simulink model "BallRegulator"  (R2026a)
settings: Solver=VariableStepAuto
libraries: fl_lib x6, nesl_utility x4, SimscapeFluids_lib x1, slpidlib x1
settings Model: Creator=lucas  LastModifiedBy=lucas

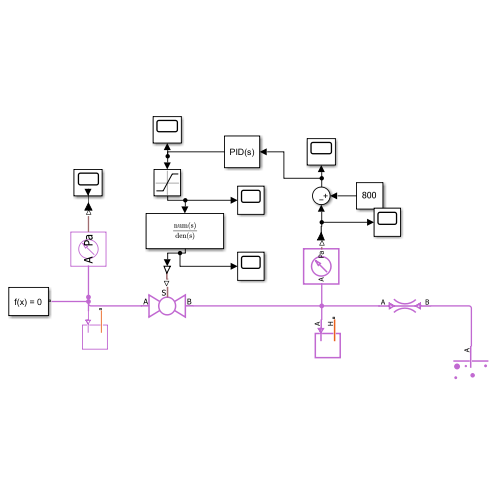
[thumbnail: Simulink's stored preview of the top-level diagram]
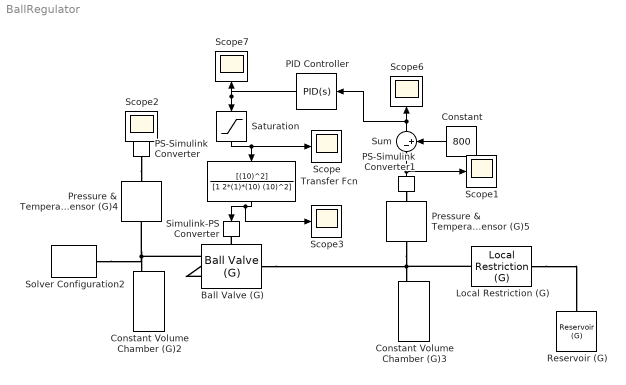
== system BallRegulator ==
  Ball Valve (G) : SimscapeFluids_lib/Gas/Valves & Orifices/Flow Control Valves/Ball Valve (G)  valve_parameterization=fluids.gas.valves_orifices.flow_control_valves.enum.OrificeParameterization.Geometry  opening_characteristic=fluids.gas.valves_orifices.flow_control_valves.enum.BallValveSpec.OverlappingCircles  Cv_max=4  rotation_Cv_TLU=pi / 2 * (0 : 0.1 : 1) rad  Cv_TLU=[1e-06, .0725, .1437, .2375, .35, .5375, .875, 1.3125, 2.125, 3.25, 4]  xT_Cv=0.7  Kv_max=3.6  rotation_Kv_TLU=pi / 2 * (0 : 0.1 : 1) rad  Kv_TLU=[1e-06, .0653, .1293, .2137, .315, .4838, .7875, 1.1813, 1.8381, 2.8112, 3.6]  xT_Kv=0.7  C_max=12 l/(bar*s)  B_crit_C=0.3  rotation_C_TLU=pi / 2 * (0 : 0.1 : 1) rad  C_TLU=[1e-05, .2175, .4312, .7125, 1.05, 1.6125, 2.625, 3.9375, 6.375, 9.75, 12] l/(bar*s)  B_crit_TLU=0.3 * ones(1, 11)  m=0.5  T_ref_C=293.15 K  rho_ref_C=1.185 kg/m^3  rotation_area_TLU=pi / 2 * (0 : 0.1 : 1) rad  area_TLU=[1e-10, 45, 90, 135, 180, 225, 270, 315, 360, 405, 450] mm^2  area_ball=pi * ((1/3) ^ 2) in^2  area=pi * ((1/2) ^ 2) in^2  Cd=0.64  leakage_fraction=1e-6  B_lam=0.999
  Constant : Constant  Value=800
  Constant Volume Chamber (G)2 : fl_lib/Gas/Elements/Constant Volume Chamber (G)  volume=0.01 m^3  num_ports=foundation.enum.num_ports.one  area_A=0.01 m^2  area_B=0.01 m^2  area_C=0.01 m^2  area_D=0.01 m^2  p_I_specify=on  p_I_priority=High  p_I=4500 psi  p_I_nominal_specify=off  p_I_nominal_value=1  p_I_nominal_unit=MPa  T_I_specify=off  T_I_priority=High  T_I=293.15 K  T_I_nominal_specify=off  T_I_nominal_value=1  T_I_nominal_unit=K  rho_I_specify=off  rho_I_priority=None  rho_I=1.2 kg/m^3  rho_I_nominal_specify=off  rho_I_nominal_value=1  rho_I_nominal_unit=kg/m^3
  Constant Volume Chamber (G)3 : fl_lib/Gas/Elements/Constant Volume Chamber (G)  volume=0.01 m^3  num_ports=foundation.enum.num_ports.one  area_A=0.01 m^2  area_B=0.01 m^2  area_C=0.01 m^2  area_D=0.01 m^2  p_I_specify=on  p_I_priority=Low  p_I=600 psi  p_I_nominal_specify=off  p_I_nominal_value=1  p_I_nominal_unit=MPa  T_I_specify=off  T_I_priority=High  T_I=293.15 K  T_I_nominal_specify=off  T_I_nominal_value=1  T_I_nominal_unit=K  rho_I_specify=off  rho_I_priority=None  rho_I=1.2 kg/m^3  rho_I_nominal_specify=off  rho_I_nominal_value=1  rho_I_nominal_unit=kg/m^3
  Local Restriction (G) : fl_lib/Gas/Elements/Local Restriction (G)  restriction_type=foundation.enum.restriction_type.fixed  restriction_area=pi * ((1/8)^2) in^2  min_area=1e-10 m^2  max_area=0.005 m^2  area=0.01 m^2  Cd=0.64  B_lam=0.999
  PID Controller : slpidlib/PID Controller  Controller=PID  Form=Parallel  TimeDomain=Continuous-time  UseExternalTs=off  SampleTime=-1  IntegratorMethod=Forward Euler  FilterMethod=Forward Euler  ControllerParametersSource=internal  P=0.005  I=0.01  UseKiTs=off  D=0.001  UseExternalDerivativeSource=off  N=100  UseFilter=on  TunerSelectOption=Transfer Function Based (PID Tuner App)  InitialConditionSource=internal  InitialConditionForIntegrator=0  InitialConditionForFilter=0  DifferentiatorICPrevScaledInput=0  ExternalReset=none  TrackingMode=off  Kt=1  LimitOutput=off  SatLimitsSource=internal  UpperSaturationLimit=inf  LowerSaturationLimit=-inf  LinearizeAsGain=on  AntiWindupMode=none  Kb=1  LimitIntegrator=off  UpperIntegratorSaturationLimit=inf  LowerIntegratorSaturationLimit=-inf  POutMin=[]  POutMax=[]  IOutMin=[]  IOutMax=[]  DOutMin=[]  DOutMax=[]  NOutMin=[]  NOutMax=[]  SumOutMin=[]  SumOutMax=[]  SaturationOutMin=[]  SaturationOutMax=[]  PParamMin=[]  PParamMax=[]  IParamMin=[]  IParamMax=[]  DParamMin=[]  DParamMax=[]  NParamMin=[]  NParamMax=[]  KbParamMin=[]  KbParamMax=[]  KtParamMin=[]  KtParamMax=[]  KbOutMin=[]  KbOutMax=[]  KtOutMin=[]  KtOutMax=[]  IntegratorOutMin=[]  IntegratorOutMax=[]  FilterOutMin=[]  FilterOutMax=[]  SumI1OutMin=[]  SumI1OutMax=[]  SumI2OutMin=[]  SumI2OutMax=[]  SumI3OutMin=[]  SumI3OutMax=[]  SumI4OutMin=[]  SumI4OutMax=[]  SumDOutMin=[]  SumDOutMax=[]  DifferentiatorOutMin=[]  DifferentiatorOutMax=[]  FilterDiffOutCoefMin=[]  FilterDiffOutCoefMax=[]  ReciprocalOutMin=[]  ReciprocalOutMax=[]  SumDenOutMin=[]  SumDenOutMax=[]  SumNumOutMin=[]  SumNumOutMax=[]  DivideOutMin=[]  DivideOutMax=[]  UdiffTsProdOutMin=[]  UdiffTsProdOutMax=[]  NTsProdOutMin=[]  NTsProdOutMax=[]  UintegralTsProdOutMin=[]  UintegralTsProdOutMax=[]  UngainTsProdOutMin=[]  UngainTsProdOutMax=[]  ClampingZeroOutDataTypeStr=Inherit: Inherit via back propagation  ClampingZeroOutMin=[]  ClampingZeroOutMax=[]  FilterDenConstantOutDataTypeStr=Inherit: Inherit via back propagation  FilterDenConstantOutMin=[]  FilterDenConstantOutMax=[]  PCopyOutDataTypeStr=Inherit: Inherit via back propagation  PCopyOutMin=[]  PCopyOutMax=[]  NCopyOutDataTypeStr=Inherit: Inherit via back propagation  NCopyOutMin=[]  NCopyOutMax=[]  IntegratorContinuousStateAttributes=''  IntegratorStateMustResolveToSignalObject=off  IntegratorRTWStateStorageClass=Auto  FilterContinuousStateAttributes=''  FilterStateMustResolveToSignalObject=off  FilterRTWStateStorageClass=Auto  ParallelPVariant=InternalParameters  IdealPVariant=Disabled  IVariant=InternalParameters  DVariant=InternalParameters  IntegratorVariant=Continuous  SatVariant=Disabled  AWVariant=Passthrough  PCopyVariant=Disabled  TRVariant=Disabled  FdbkBlocksVariant=Forward  IdealPFdbkVariant=Disabled  SatFdbkVariant=Disabled  DerivativeFilterVariant=ContFilter  NVariant=InternalParameters  NCopyVariant=Disabled  FilterICVariant=InternalICsFilter  IntegratorICVariant=InternalICs  ExternalResetVariant=Disabled  TRSumVariant=Passthrough  SumFdbkVariant=Disabled  SumVariant=Sum_PID  TsampFilterVariant=InternalTs  TsampNgainVariant=Passthrough  TsampIntegralVariant=Disabled_SignalSpec  ExternalSaturationOutDataTypeStr=Inherit: Same as second input  DerivativeSourceVariant=ErrorSignal  PreIntVariant=InternalPreInt
  PS-Simulink Converter : nesl_utility/PS-Simulink Converter  PhysicalDomain=network_engine_domain  SubClassName=ps_output  LeftPortType=input  RightPortType=output  PseudoPeriodic=off  Frequencies=[]  VectorFormat=inherit  Unit=psi  AffineConversion=off
  PS-Simulink Converter1 : nesl_utility/PS-Simulink Converter  PhysicalDomain=network_engine_domain  SubClassName=ps_output  LeftPortType=input  RightPortType=output  PseudoPeriodic=off  Frequencies=[]  VectorFormat=inherit  Unit=psi  AffineConversion=off
  Pressure & Temperature Sensor (G)4 : fl_lib/Gas/Sensors/Pressure & Temperature Sensor (G)  reference=foundation.enum.MeasurementReference.absolute  pressure=true  pressure_spec=foundation.enum.PressureMeasementSpec.Absolute  temperature=false
  Pressure & Temperature Sensor (G)5 : fl_lib/Gas/Sensors/Pressure & Temperature Sensor (G)  reference=foundation.enum.MeasurementReference.absolute  pressure=true  pressure_spec=foundation.enum.PressureMeasementSpec.Absolute  temperature=false
  Reservoir (G) : fl_lib/Gas/Elements/Reservoir (G)  pressure_input=false  pressure_spec=foundation.enum.pressure_spec.atmospheric  reservoir_pressure=0.101325 MPa  temperature_input=false  reservoir_temperature=293.15 K  area_A=0.01 m^2  input_error_spec=foundation.enum.input_range_error.warn
  Saturation : Saturate  UpperLimit=pi/2  LowerLimit=0
  Scope{,1..3,6..7} (6 alike) : Scope
      Scope settings: ActiveDisplayYMinimum=-0.73133757213653627  ActiveDisplayYMaximum=2.7321181317120371
      Scope1 settings: ActiveDisplayYMinimum=309.130990645238  ActiveDisplayYMaximum=966.57527246233519  DataLoggingVariableName=ScopeData2
      Scope2 settings: ActiveDisplayYMinimum=-3681.3578256064739  ActiveDisplayYMaximum=6147.0411122714377
      Scope3 settings: ActiveDisplayYMinimum=-0.31217932362666045  ActiveDisplayYMaximum=1.8356200833142342  DataLoggingVariableName=ScopeData3
      Scope6 settings: ActiveDisplayYMinimum=-7.853312453352288  ActiveDisplayYMaximum=318.42433199309414  DataLoggingVariableName=ScopeData6
      Scope7 settings: ActiveDisplayYMinimum=-1562.4196802548124  ActiveDisplayYMaximum=4840.2688533616483  DataLoggingVariableName=ScopeData7
  Simulink-PS Converter : nesl_utility/Simulink-PS Converter  PhysicalDomain=network_engine_domain  SubClassName=ps_input  LeftPortType=input  RightPortType=output  PseudoPeriodic=off  Frequencies=[]  NoiseDistribution=none  NoiseParameters=[]  Unit=1  AffineConversion=off  FilteringAndDerivatives=provide  SimscapeFilterOrder=1  InputFilterTimeConstant=0.001  UdotUserProvided=0
  Solver Configuration2 : nesl_utility/Solver Configuration  PhysicalDomain=network_engine_domain  SubClassName=solver  LeftPortType=input  RightPortType=generic  Tones=[]  Harmonics=[]  SimulateNoise=off  Profile=off  UseLocalSampling=off  EnableSwitchedLinearOptims=on  FrequencyDomain=off  UseCCode=off  RelTol=0.001  AbsTol=0.001  MinStep=1e-09  ToWorkspace=off  RevertToSquareIcSolve=off  NumHomotopyIterations=100  PhasorMode=off  PhasorModeNumHarmonics=1  ConsistencySolver=NEWTON_XTOL_AFTER_FTOL  CanonicalOrdering=CANONICAL  OptimizeIntermediates=OPTIMIZED  IndexReductionMethod=DerivativeReplacement  DoDC=off  ResidualTolerance=1e-09  ConsistencyTolSource=GLOBAL  ConsistencyAbsTol=0.001  ConsistencyRelTol=0.001  ConsistencyTolFactor=0.001  UseLocalSolver=off  LocalSolverChoice=NE_BACKWARD_EULER_ADVANCER  ResolveIndetEquations=on  FunctionEvalNumThread=1  LocalSolverSampleTime=0.001  DoFixedCost=off  MaxNonlinIter=3  MaxModeIter=2  ComputeImpulses=off  ImpulseIterations=2  LinearAlgebra=auto  LinearAlgebraNumThread=0  EquationFormulation=NE_TIME_EF  DelaysMemoryBudget=1024  AutomaticFiltering=on  FilteringTimeConstant=0.001  PartitionStorageMethod=AS_NEEDED  PartitionMemoryBudget=1024  PartitionMethod=ROBUST  MultibodyUseLocalSolver=off  MultibodyLocalSolverChoice=ODE1  MultibodyLocalSolverSampleTime=0.001
  Sum : Sum  Inputs=|-+
  Transfer Fcn : TransferFcn  Numerator=[(10)^2]  Denominator=[1 2*(1)*(10) (10)^2]
  wires:
  Saturation/1 -> Transfer Fcn/1, Scope/1
  Sum/1 -> PID Controller/1, Scope6/1
  PID Controller/1 -> Saturation/1, Scope7/1
  Constant/1 -> Sum/2
  PS-Simulink Converter/1 -> Scope2/1
  PS-Simulink Converter1/1 -> Sum/1, Scope1/1
  Transfer Fcn/1 -> Scope3/1, Simulink-PS Converter/1
  connections:
  Constant Volume Chamber (G)2/LConn1 -- Ball Valve (G)/LConn1 -- Solver Configuration2/RConn1 -- Pressure & Temperature Sensor (G)4/LConn1
  Ball Valve (G)/RConn1 -- Local Restriction (G)/LConn1 -- Constant Volume Chamber (G)3/LConn1 -- Pressure & Temperature Sensor (G)5/LConn1
  PS-Simulink Converter/LConn1 -- Pressure & Temperature Sensor (G)4/RConn1
  PS-Simulink Converter1/LConn1 -- Pressure & Temperature Sensor (G)5/RConn1
  Ball Valve (G)/LConn2 -- Simulink-PS Converter/RConn1
  Local Restriction (G)/RConn1 -- Reservoir (G)/LConn1
